simulink model "s_b16a4x512f"  (R2016b)
settings: Solver=VariableStepDiscrete  StartTime=0.0  StopTime=1  RelTol=1e-3
undefined symbols (not defined in the file): fft_stages, n_bits_ants, n_bits_xengs
libraries: xbsIndex_r4 x23057, casper_library_misc x150, xbsReplacements_r4 x9, casper_library_delays x8, xps_library x3
(part 80 of 210)

== system s_b16a4x512f/sys0/xeng/xeng_descramble/read_ctrl ==
  start : Inport
  Constant1 : xbsIndex_r4/Constant  const=ship_el_cnt  gui_display_data_type=Fixed-point  arith_type=Unsigned  n_bits=ceil(log2(ship_el_cnt+1))  bin_pt=0  preci_type=Single  exp_width=8  frac_width=24  explicit_period=on  period=1  equ=P=C  opselect=C  inp2=PCIN>>17  opr=+  inp1=P  carry=CIN  dbl_ovrd=off  block_type=constant
      settings: block_version=9.2.01
  Constant2 : xbsIndex_r4/Constant  const=ship_el_del  gui_display_data_type=Fixed-point  arith_type=Unsigned  n_bits=ship_el_del_bits  bin_pt=0  preci_type=Single  exp_width=8  frac_width=24  explicit_period=on  period=1  equ=P=C  opselect=C  inp2=PCIN>>17  opr=+  inp1=P  carry=CIN  dbl_ovrd=off  block_type=constant
      settings: block_version=9.2.01
  Gateway Out{1..2,4..8} (7 alike) : xbsIndex_r4/Gateway Out  inherit_from_input=off  hdl_port=off  rows=1  columns=1  UseAsDAC=off  DACChannel='1'  interface=None  automatic_assignment=on  address_offset=hex2dec('00')  intf_name=''  intf_description=''  timing_constraint=None  locs_specified=off  LOCs={}  io_standard={}  block_type=gatewayout
      settings: infoedit="Gateway out block.  Converts Xilinx fixed point inputs into ouputs of type Simulink integer, double, or fixed point.<P><P>Hardware notes:  In hardware these blocks become top level output ports or are discarded, depending on how they are configured."  xl_area=[0, 0, 0, 0, 0, 0, 0]  block_version=10.1.3
  Inverter3 : xbsIndex_r4/Inverter  en=off  latency=0  dbl_ovrd=off  block_type=inv
      settings: xl_area=[0, 0, 0, 0, 0, 0, 0]  block_version=9.2.01
  Logical1 : xbsIndex_r4/Logical  logical_function=AND  inputs=2  en=off  latency=0  precision=Full  arith_type=Unsigned  n_bits=8  bin_pt=2  align_bp=on  dbl_ovrd=off  block_type=logical
      settings: xl_area=[0, 0, 0, 0, 0, 0, 0]  block_version=9.2.01
  Logical7 : xbsIndex_r4/Logical  logical_function=OR  inputs=2  en=off  latency=0  precision=Full  arith_type=Unsigned  n_bits=8  bin_pt=2  align_bp=on  dbl_ovrd=off  block_type=logical
      settings: xl_area=[0, 0, 0, 0, 0, 0, 0]  block_version=9.2.01
  Register : xbsIndex_r4/Register  init=0  rst=on  en=on  dbl_ovrd=off  block_type=register
  Relational1 : xbsIndex_r4/Relational  mode=a<=b  op_type=Bool  en=off  latency=0  dbl_ovrd=off  block_type=relational
      settings: xl_area=[0, 0, 0, 0, 0, 0, 0]  block_version=9.2.01
  Relational3 : xbsIndex_r4/Relational  mode=a<=b  op_type=Bool  en=off  latency=0  dbl_ovrd=off  block_type=relational
      settings: xl_area=[0, 0, 0, 0, 0, 0, 0]  block_version=9.2.01
  Scope1 : Scope  NumInputPorts=7
  element : xbsIndex_r4/Counter  cnt_type=Free Running  cnt_to=demux_factor*num_elements+1  operation=Up  start_count=0  cnt_by_val=1  arith_type=Unsigned  n_bits=ceil(log2(ship_el_cnt+1))  bin_pt=0  load_pin=off  rst=on  en=on  explicit_period=off  period=1  use_behavioral_HDL=off  implementation=Fabric  use_rpm=on  dbl_ovrd=off  block_type=counter
      settings: xl_area=[0, 0, 0, 0, 0, 0, 0]  block_version=9.2.01
  ship_element_delay : xbsIndex_r4/Counter  cnt_type=Free Running  cnt_to=1  operation=Up  start_count=0  cnt_by_val=1  arith_type=Unsigned  n_bits=ship_el_del_bits  bin_pt=0  load_pin=off  rst=on  en=off  explicit_period=off  period=1  use_behavioral_HDL=off  implementation=Fabric  use_rpm=on  dbl_ovrd=off  block_type=counter
      settings: xl_area=[0, 0, 0, 0, 0, 0, 0]  block_version=9.2.01
  read_addr : Outport
  enable : Outport  Port=2
  wires:
  Relational3/1 -> Register/3, Register/1
  Inverter3/1 -> Logical1/2
  Register/1 -> Inverter3/1
  Logical1/1 -> element/2, Gateway Out1/1, enable/1, Gateway Out4/1
  Gateway Out2/1 -> Scope1/7
  Gateway Out1/1 -> Scope1/6
  Gateway Out8/1 -> Scope1/3
  Gateway Out6/1 -> Scope1/2
  Gateway Out5/1 -> Scope1/1
  Gateway Out4/1 -> Scope1/4
  Gateway Out7/1 -> Scope1/5
  Relational1/1 -> Logical1/1, Logical7/2, Gateway Out8/1
  Logical7/1 -> ship_element_delay/1
  ship_element_delay/1 -> Gateway Out6/1, Relational1/2
  Constant2/1 -> Relational1/1
  Constant1/1 -> Relational3/1
  element/1 -> Gateway Out2/1, read_addr/1, Relational3/2, Gateway Out7/1
  start/1 -> Register/2, element/1, Gateway Out5/1, Logical7/1

== system s_b16a4x512f/sys0/xeng/xeng_descramble/write_ctrl ==
  note: Lock onto start of new
      | valid window if previous
      | window was invalid
  note: negedge delay to
      | accomodate
      | a valid window followed
      | by an invalid window
  note: Flip this ordering to correct for
      | AxBx,AyBy,AyBx,AxBy ->AxBx,AyBy,AxBy,AyBx
  sync : Inport
  data_in : Inport  Port=2
  xeng_valid : Inport  Port=3
  window_valid : Inport  Port=4
  AddSub : xbsIndex_r4/AddSub  mode=Subtraction  use_carryin=off  use_carryout=off  en=off  latency=0  precision=Full  arith_type=Unsigned  n_bits=8  bin_pt=2  quantization=Truncate  overflow=Wrap  use_behavioral_HDL=on  hw_selection=Fabric  pipelined=off  use_rpm=on  dbl_ovrd=off  block_type=addsub
      settings: xl_area=[0, 0, 0, 0, 0, 0, 0]  block_version=9.2.01
  Constant : xbsIndex_r4/Constant  const=num_taps-1  gui_display_data_type=Fixed-point  arith_type=Unsigned  n_bits=taps_bits  bin_pt=0  preci_type=Single  exp_width=8  frac_width=24  explicit_period=on  period=1  equ=P=C  opselect=C  inp2=PCIN>>17  opr=+  inp1=P  carry=CIN  dbl_ovrd=off  block_type=constant
      settings: block_version=9.2.01
  Constant3 : xbsIndex_r4/Constant  const=ceil(num_validins*3/4)  gui_display_data_type=Fixed-point  arith_type=Unsigned  n_bits=validin_bits  bin_pt=0  preci_type=Single  exp_width=8  frac_width=24  explicit_period=on  period=1  equ=P=C  opselect=C  inp2=PCIN>>17  opr=+  inp1=P  carry=CIN  dbl_ovrd=off  block_type=constant
      settings: block_version=9.2.01
  Constant5 : xbsIndex_r4/Constant  const=0  gui_display_data_type=Fixed-point  arith_type=Unsigned  n_bits=taps_bits  bin_pt=0  preci_type=Single  exp_width=8  frac_width=24  explicit_period=on  period=1  equ=P=C  opselect=C  inp2=PCIN>>17  opr=+  inp1=P  carry=CIN  dbl_ovrd=off  block_type=constant
      settings: block_version=9.2.01
  Constant7 : xbsIndex_r4/Constant  const=num_taps-1  gui_display_data_type=Fixed-point  arith_type=Unsigned  n_bits=taps_bits  bin_pt=0  preci_type=Single  exp_width=8  frac_width=24  explicit_period=on  period=1  equ=P=C  opselect=C  inp2=PCIN>>17  opr=+  inp1=P  carry=CIN  dbl_ovrd=off  block_type=constant
      settings: block_version=9.2.01
  Convert : xbsIndex_r4/Convert  gui_display_data_type=Fixed-point  arith_type=Unsigned  n_bits=taps_bits+1  bin_pt=0  float_type=Single  exp_bits=8  fraction_bits=24  quantization=Truncate  overflow=Wrap  en=off  latency=0  pipeline=off  dbl_ovrd=off  block_type=convert
      settings: xl_area=[0, 0, 0, 0, 0, 0, 0]  block_version=9.2.01
  Counter2 : xbsIndex_r4/Counter  cnt_type=Count Limited  cnt_to=num_elements-1  operation=Up  start_count=pivot_pnt  cnt_by_val=1  arith_type=Unsigned  n_bits=ceil(log2(num_elements))  bin_pt=0  load_pin=off  rst=on  en=on  explicit_period=off  period=1  use_behavioral_HDL=off  implementation=Fabric  use_rpm=on  dbl_ovrd=off  block_type=counter
      settings: xl_area=[0, 0, 0, 0, 0, 0, 0]  block_version=9.2.01
  Counter3 : xbsIndex_r4/Counter  cnt_type=Count Limited  cnt_to=pivot_pnt-1  operation=Up  start_count=0  cnt_by_val=1  arith_type=Unsigned  n_bits=ceil(log2(num_elements))  bin_pt=0  load_pin=off  rst=on  en=on  explicit_period=off  period=1  use_behavioral_HDL=off  implementation=Fabric  use_rpm=on  dbl_ovrd=off  block_type=counter
      settings: xl_area=[0, 0, 0, 0, 0, 0, 0]  block_version=9.2.01
  Delay{,1..6} (7 alike) : xbsIndex_r4/Delay  rst=off  infoeditControl=Selection of Reset will increase slice count due to use of real FFs and instead of SRLs  en=off  latency=1  reg_retiming=on  dbl_ovrd=off  block_type=delay
  Gateway Out{1..8} (8 alike) : xbsIndex_r4/Gateway Out  inherit_from_input=off  hdl_port=off  rows=1  columns=1  UseAsDAC=off  DACChannel='1'  interface=None  automatic_assignment=on  address_offset=hex2dec('00')  intf_name=''  intf_description=''  timing_constraint=None  locs_specified=off  LOCs={}  io_standard={}  block_type=gatewayout
      settings: infoedit="Gateway out block.  Converts Xilinx fixed point inputs into ouputs of type Simulink integer, double, or fixed point.<P><P>Hardware notes:  In hardware these blocks become top level output ports or are discarded, depending on how they are configured."  xl_area=[0, 0, 0, 0, 0, 0, 0]  block_version=10.1.3
  Inverter{,1..3} (4 alike) : xbsIndex_r4/Inverter  en=off  latency=0  dbl_ovrd=off  block_type=inv
      settings: xl_area=[0, 0, 0, 0, 0, 0, 0]  block_version=9.2.01
  Logical{,2..3,5,7} (5 alike) : xbsIndex_r4/Logical  logical_function=AND  inputs=2  en=off  latency=0  precision=Full  arith_type=Unsigned  n_bits=8  bin_pt=2  align_bp=on  dbl_ovrd=off  block_type=logical
      settings: xl_area=[0, 0, 0, 0, 0, 0, 0]  block_version=9.2.01
  Logical1 : xbsIndex_r4/Logical  logical_function=OR  inputs=2  en=off  latency=0  precision=Full  arith_type=Unsigned  n_bits=8  bin_pt=2  align_bp=on  dbl_ovrd=off  block_type=logical
      settings: xl_area=[0, 0, 0, 0, 0, 0, 0]  block_version=9.2.01
  Logical4 : xbsIndex_r4/Logical  logical_function=AND  inputs=3  en=off  latency=0  precision=Full  arith_type=Unsigned  n_bits=8  bin_pt=2  align_bp=on  dbl_ovrd=off  block_type=logical
      settings: xl_area=[0, 0, 0, 0, 0, 0, 0]  block_version=9.2.01
  Logical6 : xbsIndex_r4/Logical  logical_function=OR  inputs=2  en=off  latency=0  precision=Full  arith_type=Unsigned  n_bits=8  bin_pt=2  align_bp=on  dbl_ovrd=off  block_type=logical
      settings: xl_area=[0, 0, 0, 0, 0, 0, 0]  block_version=9.2.01
  Mux : xbsIndex_r4/Mux  inputs=2  en=off  latency=0  precision=Full  arith_type="Signed  (2's comp)"  n_bits=8  bin_pt=2  quantization=Truncate  overflow=Wrap  dbl_ovrd=off  block_type=mux
      settings: xl_area=[0, 0, 0, 0, 0, 0, 0]  block_version=9.2.01
  Relational : xbsIndex_r4/Relational  mode=a=b  op_type=Bool  en=off  latency=0  dbl_ovrd=off  block_type=relational
      settings: xl_area=[0, 0, 0, 0, 0, 0, 0]  block_version=9.2.01
  Relational1 : xbsIndex_r4/Relational  mode=a>=b  op_type=Bool  en=off  latency=1  dbl_ovrd=off  block_type=relational
      settings: xl_area=[0, 0, 0, 0, 0, 0, 0]  block_version=9.2.01
  Relational3 : xbsIndex_r4/Relational  mode=a=b  op_type=Bool  en=off  latency=1  dbl_ovrd=off  block_type=relational
      settings: xl_area=[0, 0, 0, 0, 0, 0, 0]  block_version=9.2.01
  Relational4 : xbsIndex_r4/Relational  mode=a=b  op_type=Bool  en=off  latency=1  dbl_ovrd=off  block_type=relational
      settings: xl_area=[0, 0, 0, 0, 0, 0, 0]  block_version=9.2.01
  element_number : xbsIndex_r4/Counter  cnt_type=Count Limited  cnt_to=num_validins-1  operation=Up  start_count=0  cnt_by_val=1  arith_type=Unsigned  n_bits=validin_bits  bin_pt=0  load_pin=off  rst=on  en=on  explicit_period=off  period=1  use_behavioral_HDL=off  implementation=Fabric  use_rpm=on  dbl_ovrd=off  block_type=counter
      settings: xl_area=[0, 0, 0, 0, 0, 0, 0]  block_version=9.2.01
  line_number : xbsIndex_r4/Counter  cnt_type=Count Limited  cnt_to=num_ants-1  operation=Up  start_count=0  cnt_by_val=1  arith_type=Unsigned  n_bits=ant_bits  bin_pt=0  load_pin=off  rst=on  en=on  explicit_period=off  period=1  use_behavioral_HDL=off  implementation=Fabric  use_rpm=on  dbl_ovrd=off  block_type=counter
      settings: xl_area=[0, 0, 0, 0, 0, 0, 0]  block_version=9.2.01
  negate{1..4} (4 alike) : xbsIndex_r4/Negate  precision=User Defined  arith_type="Signed  (2's comp)"  n_bits=n_bits_xeng_out  bin_pt=0  quantization=Truncate  overflow=Wrap  en=off  latency=0  dbl_ovrd=off  block_type=negate
      negate1 settings: block_version=11.4
      negate2 settings: AttributesFormatString=num_ants=8  block_version=11.4
      negate3 settings: block_version=11.4
      negate4 settings: block_version=11.4
  negedge_delay : casper_library_misc/negedge_delay  pulse_len=ceil(num_ants/2)*acc_len
  posedge : casper_library_misc/edge_detect  edge=Rising  polarity=Active High  x_in=[0 0.08 0.08 0.16 0.16 0.24 0.24 0.32 0.32 0.4]  y_in="[-1 -1  1  1  1  1  1  1  1  1]"  x_out=[0.6 0.68 0.68 0.76 0.76 0.84 0.84 0.92 0.92 1]  y_out="[-1 -1  1  1 -1 -1 -1 -1 -1 -1]"
  posedge1 : casper_library_misc/edge_detect  edge=Rising  polarity=Active High  x_in=[0 0.08 0.08 0.16 0.16 0.24 0.24 0.32 0.32 0.4]  y_in="[-1 -1  1  1  1  1  1  1  1  1]"  x_out=[0.6 0.68 0.68 0.76 0.76 0.84 0.84 0.92 0.92 1]  y_out="[-1 -1  1  1 -1 -1 -1 -1 -1 -1]"
  remux : xbsIndex_r4/Concat  num_inputs=4  dbl_ovrd=off  block_type=concat
  repack{1..4} (4 alike) : casper_library_misc/ri_to_c
  sel_conj : xbsIndex_r4/Mux  inputs=2  en=off  latency=0  precision=Full  arith_type=Unsigned  n_bits=16  bin_pt=14  quantization=Truncate  overflow=Wrap  dbl_ovrd=off  block_type=mux
  slice1 : xbsIndex_r4/Slice  nbits=2*n_bits_xeng_out  boolean_output=off  mode=Lower Bit Location + Width  bit1=0  base1=MSB of Input  bit0=2*n_bits_xeng_out*3  base0=LSB of Input  dbl_ovrd=off  block_type=slice
  slice2 : xbsIndex_r4/Slice  nbits=2*n_bits_xeng_out  boolean_output=off  mode=Lower Bit Location + Width  bit1=0  base1=MSB of Input  bit0=4*n_bits_xeng_out  base0=LSB of Input  dbl_ovrd=off  block_type=slice
  slice3 : xbsIndex_r4/Slice  nbits=2*n_bits_xeng_out  boolean_output=off  mode=Lower Bit Location + Width  bit1=0  base1=MSB of Input  bit0=2*n_bits_xeng_out  base0=LSB of Input  dbl_ovrd=off  block_type=slice
  slice4 : xbsIndex_r4/Slice  nbits=2*n_bits_xeng_out  boolean_output=off  mode=Lower Bit Location + Width  bit1=0  base1=MSB of Input  bit0=0  base0=LSB of Input  dbl_ovrd=off  block_type=slice
  tap_number : xbsIndex_r4/Counter  cnt_type=Count Limited  cnt_to=num_taps-1  operation=Up  start_count=0  cnt_by_val=1  arith_type=Unsigned  n_bits=taps_bits  bin_pt=0  load_pin=off  rst=on  en=on  explicit_period=off  period=1  use_behavioral_HDL=off  implementation=Fabric  use_rpm=on  dbl_ovrd=off  block_type=counter
      settings: xl_area=[0, 0, 0, 0, 0, 0, 0]  block_version=9.2.01
  unpack{1..4} (4 alike) : casper_library_misc/c_to_ri  n_bits=n_bits_xeng_out  bin_pt=0
      settings: AttributesFormatString=25_0 r/i
  wr_ctl_debug : Scope  NumInputPorts=8
  start_readout : Outport
  write_addr : Outport  Port=2
  data_out : Outport  Port=3
  enable : Outport  Port=4
  wires:
  Delay3/1 -> [data_in]
  data_in/1 -> Delay3/1
  Delay1/1 -> [valid_in]
  sync/1 -> Delay/1
  Logical1/1 -> [rst_in]
  xeng_valid/1 -> Logical2/2
  posedge/1 -> Logical1/2
  Delay/1 -> Logical1/1
  window_valid/1 -> negedge_delay/1, posedge/1
  Logical2/1 -> Delay1/1
  negedge_delay/1 -> Logical2/1
  [data_in] -> Delay6/1
  [last_triangle] -> sel_conj/1
  repack4/1 -> remux/3
  repack3/1 -> remux/4
  Delay6/1 -> sel_conj/2, slice1/1, slice2/1, slice3/1, slice4/1
  sel_conj/1 -> data_out/1
  remux/1 -> sel_conj/3
  slice1/1 -> unpack1/1
  unpack1/1 -> repack1/1
  unpack1/2 -> negate1/1
  negate1/1 -> repack1/2
  repack1/1 -> remux/1
  slice2/1 -> unpack2/1
  unpack2/1 -> repack2/1
  unpack2/2 -> negate2/1
  negate2/1 -> repack2/2
  repack2/1 -> remux/2
  slice3/1 -> unpack3/1
  unpack3/1 -> repack3/1
  unpack3/2 -> negate3/1
  negate3/1 -> repack3/2
  slice4/1 -> unpack4/1
  unpack4/1 -> repack4/1
  unpack4/2 -> negate4/1
  negate4/1 -> repack4/2
  Delay2/1 -> [pos_cnt]
  posedge1/1 -> start_readout/1
  Relational/1 -> Logical/1, Logical6/1
  [valid_in] -> Logical6/2
  [valid_in] -> Logical/2
  [valid_in] -> element_number/2
  Delay5/1 -> [rst]
  [valid_in] -> Delay4/1
  [rst_in] -> Delay5/1
  Delay4/1 -> [valid]
  Constant7/1 -> AddSub/1
  Logical6/1 -> tap_number/2
  Constant3/1 -> Relational3/2
  element_number/1 -> Delay2/1, Relational3/1
  Logical/1 -> line_number/2
  line_number/1 -> AddSub/2
  Inverter/1 -> Logical3/2, [last_triangle]
  Convert/1 -> Relational1/1
  Relational1/1 -> Inverter/1
  Constant/1 -> Relational/1
  AddSub/1 -> Relational1/2
  tap_number/1 -> Relational/2, Relational4/2, Convert/1
  Gateway Out7/1 -> wr_ctl_debug/5
  Gateway Out4/1 -> wr_ctl_debug/4
  Gateway Out5/1 -> wr_ctl_debug/1
  Gateway Out6/1 -> wr_ctl_debug/2
  Gateway Out8/1 -> wr_ctl_debug/3
  Gateway Out1/1 -> wr_ctl_debug/6
  Gateway Out2/1 -> wr_ctl_debug/7
  [rst_in] -> tap_number/1
  [rst_in] -> line_number/1
  [rst_in] -> element_number/1
  [rst] -> Gateway Out5/1
  [last_triangle] -> Gateway Out4/1
  Constant5/1 -> Relational4/1
  [pos_cnt] -> Gateway Out1/1
  Relational4/1 -> Logical3/1
  Logical3/1 -> [blank_it]
  [blank_it] -> Inverter1/1
  [last_triangle] -> Logical4/1
  Inverter1/1 -> Logical4/2
  Logical4/1 -> Counter2/2
  Counter2/1 -> Mux/3, Gateway Out7/1
  Counter3/1 -> Mux/2
  [rst] -> Counter2/1
  [last_triangle] -> Mux/1
  Mux/1 -> write_addr/1, Gateway Out2/1
  [last_triangle] -> Inverter2/1
  [rst] -> Counter3/1
  Logical5/1 -> Counter3/2
  [valid] -> Logical4/3
  [valid] -> Logical5/1
  Inverter2/1 -> Logical5/2
  [blank_it] -> Inverter3/1
  Inverter3/1 -> Logical7/1
  [valid] -> Logical7/2
  Gateway Out3/1 -> wr_ctl_debug/8
  Logical7/1 -> enable/1, Gateway Out3/1
  Relational3/1 -> posedge1/1
  [valid] -> Gateway Out8/1
  [blank_it] -> Gateway Out6/1

== system s_b16a4x512f/sys0/xeng/xeng_descramble/x_cast ==
  in : Inport
  Concat : xbsIndex_r4/Concat  num_inputs=8  dbl_ovrd=off  block_type=concat
      settings: block_version=9.2.01
  Convert{,1..7} (8 alike) : xbsIndex_r4/Convert  gui_display_data_type=Fixed-point  arith_type="Signed  (2's comp)"  n_bits=n_bits_out  bin_pt=fix_pnt_pos  float_type=Single  exp_bits=8  fraction_bits=24  quantization=Truncate  overflow=Wrap  en=off  latency=0  pipeline=off  dbl_ovrd=off  block_type=convert
      settings: block_version=10.1.3
  Slice : xbsIndex_r4/Slice  nbits=n_bits_in  boolean_output=off  mode=Lower Bit Location + Width  bit1=0  base1=MSB of Input  bit0=bit_offsets(1)*n_bits_in  base0=LSB of Input  dbl_ovrd=off  block_type=slice
      settings: infoedit="Extracts a given range of bits from each input sample and presents it at the output.  The output type is ordinarily unsigned with binary point at zero, but can be Boolean when the slice is one bit wide.<P><P>Hardware notes: In hardware this block costs nothing."  block_version=10.1.3
  Slice1 : xbsIndex_r4/Slice  nbits=n_bits_in  boolean_output=off  mode=Lower Bit Location + Width  bit1=0  base1=MSB of Input  bit0=bit_offsets(2)*n_bits_in  base0=LSB of Input  dbl_ovrd=off  block_type=slice
      settings: infoedit="Extracts a given range of bits from each input sample and presents it at the output.  The output type is ordinarily unsigned with binary point at zero, but can be Boolean when the slice is one bit wide.<P><P>Hardware notes: In hardware this block costs nothing."  block_version=10.1.3
  Slice2 : xbsIndex_r4/Slice  nbits=n_bits_in  boolean_output=off  mode=Lower Bit Location + Width  bit1=0  base1=MSB of Input  bit0=bit_offsets(3)*n_bits_in  base0=LSB of Input  dbl_ovrd=off  block_type=slice
      settings: infoedit="Extracts a given range of bits from each input sample and presents it at the output.  The output type is ordinarily unsigned with binary point at zero, but can be Boolean when the slice is one bit wide.<P><P>Hardware notes: In hardware this block costs nothing."  block_version=10.1.3
  Slice3 : xbsIndex_r4/Slice  nbits=n_bits_in  boolean_output=off  mode=Lower Bit Location + Width  bit1=0  base1=MSB of Input  bit0=bit_offsets(4)*n_bits_in  base0=LSB of Input  dbl_ovrd=off  block_type=slice
      settings: infoedit="Extracts a given range of bits from each input sample and presents it at the output.  The output type is ordinarily unsigned with binary point at zero, but can be Boolean when the slice is one bit wide.<P><P>Hardware notes: In hardware this block costs nothing."  block_version=10.1.3
  Slice4 : xbsIndex_r4/Slice  nbits=n_bits_in  boolean_output=off  mode=Lower Bit Location + Width  bit1=0  base1=MSB of Input  bit0=bit_offsets(5)*n_bits_in  base0=LSB of Input  dbl_ovrd=off  block_type=slice
      settings: infoedit="Extracts a given range of bits from each input sample and presents it at the output.  The output type is ordinarily unsigned with binary point at zero, but can be Boolean when the slice is one bit wide.<P><P>Hardware notes: In hardware this block costs nothing."  block_version=10.1.3
  Slice5 : xbsIndex_r4/Slice  nbits=n_bits_in  boolean_output=off  mode=Lower Bit Location + Width  bit1=0  base1=MSB of Input  bit0=bit_offsets(6)*n_bits_in  base0=LSB of Input  dbl_ovrd=off  block_type=slice
      settings: infoedit="Extracts a given range of bits from each input sample and presents it at the output.  The output type is ordinarily unsigned with binary point at zero, but can be Boolean when the slice is one bit wide.<P><P>Hardware notes: In hardware this block costs nothing."  block_version=10.1.3
  Slice6 : xbsIndex_r4/Slice  nbits=n_bits_in  boolean_output=off  mode=Lower Bit Location + Width  bit1=0  base1=MSB of Input  bit0=bit_offsets(7)*n_bits_in  base0=LSB of Input  dbl_ovrd=off  block_type=slice
      settings: infoedit="Extracts a given range of bits from each input sample and presents it at the output.  The output type is ordinarily unsigned with binary point at zero, but can be Boolean when the slice is one bit wide.<P><P>Hardware notes: In hardware this block costs nothing."  block_version=10.1.3
  Slice7 : xbsIndex_r4/Slice  nbits=n_bits_in  boolean_output=off  mode=Lower Bit Location + Width  bit1=0  base1=MSB of Input  bit0=bit_offsets(8)*n_bits_in  base0=LSB of Input  dbl_ovrd=off  block_type=slice
      settings: infoedit="Extracts a given range of bits from each input sample and presents it at the output.  The output type is ordinarily unsigned with binary point at zero, but can be Boolean when the slice is one bit wide.<P><P>Hardware notes: In hardware this block costs nothing."  block_version=10.1.3
  force_re{,1,4,6,8,10,12,14} (8 alike) : xbsIndex_r4/Reinterpret  force_arith_type=on  arith_type="Signed  (2's comp)"  force_bin_pt=on  bin_pt=fix_pnt_pos  block_type=reinterpret
      settings: infoedit="Changes signal type without altering the binary representation.   You can changed the signal between signed and unsigned, and relocate the binary point.<P><P>Hardware notes: In hardware this block costs nothing.<P><P>Example:  Suppose the input is 6 bits wide, signed, with 2 fractional bits, and the output is forced to unsigned with 0 fractional bits.  Then an input of -2.0 (1110.00 in binary 2's complement) becomes an output of 56 (111000 in binary)."  block_version=9.1.01
  force_re{2..3,5,7,9,11,13,15} (8 alike) : xbsIndex_r4/Reinterpret  force_arith_type=on  arith_type=Unsigned  force_bin_pt=on  bin_pt=0  block_type=reinterpret
      settings: infoedit="Changes signal type without altering the binary representation.   You can changed the signal between signed and unsigned, and relocate the binary point.<P><P>Hardware notes: In hardware this block costs nothing.<P><P>Example:  Suppose the input is 6 bits wide, signed, with 2 fractional bits, and the output is forced to unsigned with 0 fractional bits.  Then an input of -2.0 (1110.00 in binary 2's complement) becomes an output of 56 (111000 in binary)."  block_version=9.1.01
  out : Outport
  wires:
  force_re15/1 -> Concat/8
  force_re13/1 -> Concat/7
  force_re11/1 -> Concat/6
  force_re9/1 -> Concat/5
  force_re7/1 -> Concat/4
  force_re5/1 -> Concat/3
  Slice7/1 -> force_re14/1
  force_re14/1 -> Convert7/1
  Convert7/1 -> force_re15/1
  Slice6/1 -> force_re12/1
  force_re12/1 -> Convert6/1
  Convert6/1 -> force_re13/1
  Slice5/1 -> force_re10/1
  force_re10/1 -> Convert5/1
  Convert5/1 -> force_re11/1
  Slice4/1 -> force_re8/1
  force_re8/1 -> Convert4/1
  Convert4/1 -> force_re9/1
  Slice3/1 -> force_re6/1
  force_re6/1 -> Convert3/1
  Convert3/1 -> force_re7/1
  Slice2/1 -> force_re4/1
  force_re4/1 -> Convert2/1
  Convert2/1 -> force_re5/1
  force_re3/1 -> Concat/2
  Slice1/1 -> force_re1/1
  Concat/1 -> out/1
  in/1 -> Slice1/1, Slice2/1, Slice3/1, Slice4/1, Slice5/1, Slice7/1, Slice6/1, Slice/1
  Slice/1 -> force_re/1
  force_re1/1 -> Convert1/1
  force_re/1 -> Convert/1
  Convert1/1 -> force_re3/1
  Convert/1 -> force_re2/1
  force_re2/1 -> Concat/1

== system s_b16a4x512f/sys1/bf/fbf/apply_beam_weights ==
  note: The same coefficient
      | is kept for each 'stack'
      | of input values
  note: Xilinx addresses words in a compound
      | word as 0 in the LS word. We want it
      | the other way so we reorder the data
      | on the way in and then undo the
      | reordering on the way out again
  synci : Inport
  din : Inport  Port=2
  den : Inport  Port=3
  misci : Inport  Port=4
  index : Inport  Port=5
  vali : Inport  Port=6
  we : Inport  Port=7
  Concat : xbsIndex_r4/Concat  num_inputs=3  dbl_ovrd=off  block_type=concat
  Constant1 : xbsIndex_r4/Constant  const=0  gui_display_data_type=Fixed-point  arith_type=Boolean  n_bits=1  bin_pt=0  preci_type=Single  exp_width=8  frac_width=24  explicit_period=off  period=1  equ=P=C  opselect=C  inp2=PCIN>>17  opr=+  inp1=P  carry=CIN  dbl_ovrd=off  block_type=constant
      settings: block_version=11.4
  Slice : xbsIndex_r4/Slice  nbits=1  boolean_output=on  mode=Upper Bit Location + Width  bit1=-1  base1=MSB of Input  bit0=0  base0=LSB of Input  dbl_ovrd=off  block_type=slice
  Slice1 : xbsIndex_r4/Slice  nbits=1  boolean_output=off  mode=Two Bit Locations  bit1=-2  base1=MSB of Input  bit0=0  base0=LSB of Input  dbl_ovrd=off  block_type=slice
  Slice2 : xbsIndex_r4/Slice  nbits=1  boolean_output=on  mode=Upper Bit Location + Width  bit1=0  base1=MSB of Input  bit0=0  base0=LSB of Input  dbl_ovrd=off  block_type=slice
  add_gen : xbsIndex_r4/Counter  cnt_type=Free Running  cnt_to=Inf  operation=Up  start_count=0  cnt_by_val=1  arith_type=Unsigned  n_bits=vec_bits+stack_bits  bin_pt=0  load_pin=off  rst=on  en=on  explicit_period=on  period=1  use_behavioral_HDL=off  implementation=Fabric  dbl_ovrd=off  block_type=counter
      settings: block_version=11.4
  bus_convert : Subsystem  AncestorBlock=casper_library_bus/bus_convert  mask(bus_convert){n_bits_in=repmat(n_bits_coeff+n_bits_in+1, 1, 2^stream_bits), bin_pt_in=bin_pt_coeff+bin_pt_in, cmplx=on, n_bits_out=n_bits_out, bin_pt_out=bin_pt_out, quantization=quantization, overflow=overflow, latency=conv_latency, of=off, misc=on}
      mask prompts: n_bits_in "input bit widths"; bin_pt_in "input binary points"; cmplx "input complex"; n_bits_out "output bit widths"; bin_pt_out "output binary points"; quantization "quantization strategy (Truncate=0, Round  (unbiased: +/- Inf)=1, Round (unbiased: Even Values)=2)"; overflow "overflow strategy (Wrap=0, Saturate=1, Flag as error=2)"; of "overflow indication"; misc "misc support"
      mask help: Convert components of busses
      mask init: same as s_b16a4x512f/sys0/31->32
  bus_mult : Subsystem  AncestorBlock=casper_library_bus/bus_mult  mask(bus_mult){n_bits_a=repmat(n_bits_in, 1, 2^stream_bits), bin_pt_a=bin_pt_in, type_a=type_in, cmplx_a=on, n_bits_b=repmat(n_bits_coeff, 1, 2^stream_bits), bin_pt_b=bin_pt_coeff, type_b=type_coeff, cmplx_b=off, n_bits_out=n_bits_coeff+n_bits_in+1, bin_pt_out=bin_pt_coeff+bin_pt_in, type_out=type_out, quantization=0, overflow=0, mult_latency=mult_latency, add_latency=2, conv_latency=0, max_fanout=2, fan_latency=1, multiplier_implementation=embedded multiplier core, misc=on}
      mask prompts: n_bits_a "a input bit widths"; bin_pt_a "a input binary points"; type_a "a input type (Unsigned=0, Signed=1)"; cmplx_a "a input complex"; n_bits_b "b input bit widths"; bin_pt_b "b input binary points"; type_b "b input type (Unsigned=0, Signed=1)"; cmplx_b "b input complex"; n_bits_out "output bit widths"; bin_pt_out "output binary points"; type_out "output type (Unsigned=0, Signed=1)"; quantization "quantization strategy (Truncate=0, Round  (unbiased: +/- Inf)=1)"; overflow "overflow strategy (Wrap=0, Saturate=1, Flag as error=2)"; mult_latency "multiplier latency"; add_latency "adder latency"; conv_latency "convert latency"; max_fanout "limit fanout to ?"; fan_latency "fanout register latency"; multiplier_implementation "multiplier implementation"; misc "misc support"
      mask help: Multiply components of two busses
      mask init: same as s_b16a4x512f/sys0/bf/fbf/apply_beam_weights/bus_mult
      mask TypeOptions multiplier_implementation: behavioral HDL | standard core | embedded multiplier core
  coeffs : xbsIndex_r4/Dual Port RAM  depth=2^(vec_bits+stream_bits)  initVector=repmat(real(init_val)*2^(bin_pt_coeff),1,2^(vec_bits+stream_bits))  distributed_mem=Block RAM  init_a=0  init_b=0  rst_a=off  rst_b=off  en_a=off  en_b=off  latency=bram_latency  write_mode_A=Read After Write  write_mode_B=Read After Write  optimize=Area  dbl_ovrd=off  block_type=dpram
      settings: block_version=11.4
  ddin : xbsIndex_r4/Delay  rst=off  infoeditControl=Selection of Reset will increase slice count due to use of real FFs and instead of SRLs  en=off  latency=bram_latency  reg_retiming=off  dbl_ovrd=off  block_type=delay
      settings: block_version=11.4
  ddin1 : xbsIndex_r4/Delay  rst=off  infoeditControl=Selection of Reset will increase slice count due to use of real FFs and instead of SRLs  en=off  latency=bram_latency  reg_retiming=off  dbl_ovrd=off  block_type=delay
      settings: block_version=11.4
  dinb : xbsIndex_r4/Constant  const=0  gui_display_data_type=Fixed-point  arith_type=Unsigned  n_bits=n_bits_coeff*2^stream_bits  bin_pt=0  preci_type=Single  exp_width=8  frac_width=24  explicit_period=off  period=1  equ=P=C  opselect=C  inp2=PCIN>>17  opr=+  inp1=P  carry=CIN  dbl_ovrd=off  block_type=constant
      settings: block_version=11.4
  munge_in : Subsystem  AncestorBlock=casper_library_flow_control/munge  mask(munge){divisions=2^stream_bits, div_size=repmat(n_bits_in*2, 1, 2^stream_bits), order=max(0,2^stream_bits-1):-1:0, arith_type_out=Unsigned, bin_pt_out=0}
      mask prompts: divisions "Number of divisions"; div_size "Division size (bits)"; order "Division packing order"; arith_type_out "Output arithmetic type"; bin_pt_out "Output binary point"
      mask help: Splits an input bus into the specified number of divisions and then recombines them in the order specified (most significant division = 0,least = number divisions-1)
      mask init:
      | munge_init(gcb, ...
      |     'divisions', divisions, ...
      |     'div_size', div_size, ...
      |     'order', order, ...
      |     'arith_type_out', arith_type_out, ...
      |     'bin_pt_out', bin_pt_out);
      settings: AttributesFormatString=|
      | split:[16 16]
      | join:[1 0]
      | Unsigned [32,0]
      mask TypeOptions arith_type_out: Unsigned | Signed  (2's comp) | Floating-point
  munge_out : Subsystem  AncestorBlock=casper_library_flow_control/munge  mask(munge){divisions=2^stream_bits, div_size=repmat(n_bits_out*2, 1, 2^stream_bits), order=max(0,2^stream_bits-1):-1:0, arith_type_out=Unsigned, bin_pt_out=0}
      mask prompts: divisions "Number of divisions"; div_size "Division size (bits)"; order "Division packing order"; arith_type_out "Output arithmetic type"; bin_pt_out "Output binary point"
      mask help: Splits an input bus into the specified number of divisions and then recombines them in the order specified (most significant division = 0,least = number divisions-1)
      mask init:
      | munge_init(gcb, ...
      |     'divisions', divisions, ...
      |     'div_size', div_size, ...
      |     'order', order, ...
      |     'arith_type_out', arith_type_out, ...
      |     'bin_pt_out', bin_pt_out);
      settings: AttributesFormatString=|
      | split:[50 50]
      | join:[1 0]
      | Unsigned [100,0]
      mask TypeOptions arith_type_out: Unsigned | Signed  (2's comp) | Floating-point
  vector : xbsIndex_r4/Slice  nbits=vec_bits  boolean_output=off  mode=Lower Bit Location + Width  bit1=0  base1=MSB of Input  bit0=stack_bits  base0=LSB of Input  dbl_ovrd=off  block_type=slice
  we_slice : xbsIndex_r4/Slice  nbits=1  boolean_output=on  mode=Lower Bit Location + Width  bit1=0  base1=MSB of Input  bit0=0  base0=LSB of Input  dbl_ovrd=off  block_type=slice
  synco : Outport
  dout : Outport  Port=2
  eno : Outport  Port=3
  misco : Outport  Port=4
  valo : Outport  Port=5
  wires:
  add_gen/1 -> vector/1
  vector/1 -> coeffs/4
  dinb/1 -> coeffs/5
  we_slice/1 -> coeffs/3
  Constant1/1 -> coeffs/6
  coeffs/1 -> valo/1
  index/1 -> coeffs/1
  den/1 -> add_gen/2, Concat/2
  din/1 -> ddin/1
  we/1 -> we_slice/1
  synci/1 -> Concat/1, add_gen/1
  ddin/1 -> munge_in/1(din)
  coeffs/2 -> bus_mult/2(b)
  Concat/1 -> ddin1/1
  ddin1/1 -> bus_mult/3(misci)
  Slice/1 -> eno/1
  Slice1/1 -> misco/1
  bus_mult/1(a*b) -> bus_convert/1(din)
  bus_mult/2(misco) -> bus_convert/2(misci)
  bus_convert/1(dout) -> munge_out/1(din)
  bus_convert/2(misco) -> Slice1/1, Slice2/1, Slice/1
  misci/1 -> Concat/3
  Slice2/1 -> synco/1
  vali/1 -> coeffs/2
  munge_in/1(dout) -> bus_mult/1(a)
  munge_out/1(dout) -> dout/1

== system s_b16a4x512f/sys1/bf/fbf/bus_expand ==
  bus_in : Inport
  reinterpret{1..4} (4 alike) : xbsIndex_r4/Reinterpret  force_arith_type=on  arith_type="Signed  (2's comp)"  force_bin_pt=on  bin_pt=7  block_type=reinterpret
      settings: infoedit="Changes signal type without altering the binary representation.   You can changed the signal between signed and unsigned, and relocate the binary point.<br><br>Hardware notes: In hardware this block costs nothing.<br><br>Example:  Suppose the input is 6 bits wide, signed, with 2 fractional bits, and the output is forced to unsigned with 0 fractional bits.  Then an input of -2.0 (1110.00 in binary 2's complement) becomes an output of 56 (111000 in binary)."
  slice1 : xbsIndex_r4/Slice  nbits=8  boolean_output=off  mode=Upper Bit Location + Width  bit1=-24  base1=MSB of Input  bit0=0  base0=LSB of Input  dbl_ovrd=off  block_type=slice
  slice2 : xbsIndex_r4/Slice  nbits=8  boolean_output=off  mode=Upper Bit Location + Width  bit1=-16  base1=MSB of Input  bit0=0  base0=LSB of Input  dbl_ovrd=off  block_type=slice
  slice3 : xbsIndex_r4/Slice  nbits=8  boolean_output=off  mode=Upper Bit Location + Width  bit1=-8  base1=MSB of Input  bit0=0  base0=LSB of Input  dbl_ovrd=off  block_type=slice
  slice4 : xbsIndex_r4/Slice  nbits=8  boolean_output=off  mode=Upper Bit Location + Width  bit1=0  base1=MSB of Input  bit0=0  base0=LSB of Input  dbl_ovrd=off  block_type=slice
  msb_out4 : Outport
  out3 : Outport  Port=2
  out2 : Outport  Port=3
  lsb_out1 : Outport  Port=4
  wires:
  bus_in/1 -> slice4/1, slice3/1, slice2/1, slice1/1
  slice4/1 -> reinterpret4/1
  reinterpret4/1 -> msb_out4/1
  slice3/1 -> reinterpret3/1
  reinterpret3/1 -> out3/1
  slice2/1 -> reinterpret2/1
  reinterpret2/1 -> out2/1
  slice1/1 -> reinterpret1/1
  reinterpret1/1 -> lsb_out1/1

== system s_b16a4x512f/sys1/bf/fbf/bus_expand1 ==
  bus_in : Inport
  reinterpret{1..4} (4 alike) : xbsIndex_r4/Reinterpret  force_arith_type=on  arith_type="Signed  (2's comp)"  force_bin_pt=on  bin_pt=16  block_type=reinterpret
      settings: infoedit="Changes signal type without altering the binary representation.   You can changed the signal between signed and unsigned, and relocate the binary point.<br><br>Hardware notes: In hardware this block costs nothing.<br><br>Example:  Suppose the input is 6 bits wide, signed, with 2 fractional bits, and the output is forced to unsigned with 0 fractional bits.  Then an input of -2.0 (1110.00 in binary 2's complement) becomes an output of 56 (111000 in binary)."
  slice1 : xbsIndex_r4/Slice  nbits=25  boolean_output=off  mode=Upper Bit Location + Width  bit1=-75  base1=MSB of Input  bit0=0  base0=LSB of Input  dbl_ovrd=off  block_type=slice
  slice2 : xbsIndex_r4/Slice  nbits=25  boolean_output=off  mode=Upper Bit Location + Width  bit1=-50  base1=MSB of Input  bit0=0  base0=LSB of Input  dbl_ovrd=off  block_type=slice
  slice3 : xbsIndex_r4/Slice  nbits=25  boolean_output=off  mode=Upper Bit Location + Width  bit1=-25  base1=MSB of Input  bit0=0  base0=LSB of Input  dbl_ovrd=off  block_type=slice
  slice4 : xbsIndex_r4/Slice  nbits=25  boolean_output=off  mode=Upper Bit Location + Width  bit1=0  base1=MSB of Input  bit0=0  base0=LSB of Input  dbl_ovrd=off  block_type=slice
  msb_out4 : Outport
  out3 : Outport  Port=2
  out2 : Outport  Port=3
  lsb_out1 : Outport  Port=4
  wires:
  bus_in/1 -> slice4/1, slice3/1, slice2/1, slice1/1
  slice4/1 -> reinterpret4/1
  reinterpret4/1 -> msb_out4/1
  slice3/1 -> reinterpret3/1
  reinterpret3/1 -> out3/1
  slice2/1 -> reinterpret2/1
  reinterpret2/1 -> out2/1
  slice1/1 -> reinterpret1/1
  reinterpret1/1 -> lsb_out1/1

== system s_b16a4x512f/sys1/bf/fbf/combine ==
  note: *  accumulator that takes values for all
      | beams for bunch of time for associated antenna
      | * outputs values when all antennae
      | accounted for
      | * excludes if bad bit high
  synci : Inport
  data : Inport  Port=2
  den : Inport  Port=3
  bad : Inport  Port=4
  timei : Inport  Port=5
  misci : Inport  Port=6
  Concat : xbsIndex_r4/Concat  num_inputs=2  dbl_ovrd=off  block_type=concat
  acc : Subsystem  mask{stream_bits=stream_bits, stack_bits=stack_bits, n_bits_in=n_bits_in, bin_pt_in=bin_pt_in, n_bits_accum=n_bits_accum, bram_latency=bram_latency, add_latency=add_latency}
      mask prompts: stream_bits "input streams (2^?)"; stack_bits "stacking factor (2^?)"; n_bits_in "data bits in"; bin_pt_in "binary point in"; n_bits_accum "accumulator bits"; bram_latency "bram latency"; add_latency "add latency"
      mask init: same as s_b16a4x512f/sys0/bf/fbf/combine/acc
  acc_ctrl : Subsystem  mask{ant_bits=ant_bits, stream_bits=stream_bits, freq_bits=freq_bits, stack_bits=stack_bits, bram_latency=bram_latency}
      mask prompts: ant_bits "antennas (2^?)"; stream_bits "input streams (2^?)"; freq_bits "frequencies (2^?)"; stack_bits "stacking factor (2^?)"; bram_latency "bram latency"
  misc_slc : xbsIndex_r4/Slice  nbits=0  boolean_output=off  mode=Two Bit Locations  bit1=-timestamp_bits  base1=MSB of Input  bit0=0  base0=LSB of Input  dbl_ovrd=off  block_type=slice
  time_slc : xbsIndex_r4/Slice  nbits=timestamp_bits  boolean_output=off  mode=Upper Bit Location + Width  bit1=0  base1=MSB of Input  bit0=0  base0=LSB of Input  dbl_ovrd=off  block_type=slice
  synco : Outport
  sum : Outport  Port=2
  eno : Outport  Port=3
  timeo : Outport  Port=4
  misco : Outport  Port=5
  wires:
  acc/1(synco) -> synco/1
  acc_ctrl/1(synco) -> acc/1(synci)
  misc_slc/1 -> misco/1
  time_slc/1 -> timeo/1
  acc/4(misc_o) -> misc_slc/1, time_slc/1
  Concat/1 -> acc/6(misc_in)
  acc_ctrl/7(misco) -> Concat/2
  acc_ctrl/6(timeo) -> Concat/1
  acc_ctrl/5(dump) -> acc/5(dump)
  acc_ctrl/4(dvalid) -> acc/4(dvalid)
  bad/1 -> acc_ctrl/4(badi)
  timei/1 -> acc_ctrl/5(timei)
  acc_ctrl/3(en) -> acc/3(en)
  acc_ctrl/2(dout) -> acc/2(dat)
  synci/1 -> acc_ctrl/1(synci)
  den/1 -> acc_ctrl/3(den)
  acc/2(dato) -> sum/1
  data/1 -> acc_ctrl/2(din)
  acc/3(valid) -> eno/1
  misci/1 -> acc_ctrl/6(misci)

== system s_b16a4x512f/sys1/bf/fbf/duplicate ==
  synci : Inport
  eni : Inport  Port=2
  di : Inport  Port=3
  badi : Inport  Port=4
  timei : Inport  Port=5
  misci : Inport  Port=6
  sim_ld : Inport  Port=7
  sim_type : Inport  Port=8
  Convert1 : xbsIndex_r4/Convert  gui_display_data_type=Fixed-point  arith_type=Unsigned  n_bits=n_bits_in*2  bin_pt=0  float_type=Single  exp_bits=8  fraction_bits=24  quantization=Truncate  overflow=Wrap  en=off  latency=0  pipeline=off  dbl_ovrd=off  block_type=convert
      settings: block_version=11.4
  Counter : xbsIndex_r4/Counter  cnt_type=Free Running  cnt_to=inf  operation=Up  start_count=0  cnt_by_val=1  arith_type="Signed  (2's comp)"  n_bits=stack_bits+ant_bits+freq_bits  bin_pt=0  load_pin=off  rst=on  en=on  explicit_period=on  period=1  use_behavioral_HDL=off  implementation=Fabric  dbl_ovrd=off  block_type=counter
      settings: block_version=11.4
  Delay{,1..3,5} (5 alike) : xbsIndex_r4/Delay  rst=off  infoeditControl=Selection of Reset will increase slice count due to use of real FFs and instead of SRLs  en=off  latency=1  reg_retiming=off  dbl_ovrd=off  block_type=delay
      Delay settings: infoedit=Hardware notes: A delay line is a chain, each link of which is an SRL16 or SRL32 followed by a flip-flop.  block_version=11.4
      Delay1 settings: block_version=11.4
      Delay2 settings: block_version=11.4
      Delay3 settings: block_version=11.4
      Delay5 settings: block_version=11.4
  Mux : xbsIndex_r4/Mux  inputs=2  en=off  latency=1  precision=Full  arith_type=Unsigned  n_bits=16  bin_pt=14  quantization=Truncate  overflow=Wrap  dbl_ovrd=off  block_type=mux
      settings: block_version=11.4
  Register1 : xbsIndex_r4/Register  init=0  rst=off  en=on  dbl_ovrd=off  block_type=register
      settings: block_version=11.4
  Slice : xbsIndex_r4/Slice  nbits=freq_bits  boolean_output=off  mode=Upper Bit Location + Width  bit1=0  base1=MSB of Input  bit0=0  base0=LSB of Input  dbl_ovrd=off  block_type=slice
  beam_replicate : Subsystem  AncestorBlock=casper_library_bus/bus_replicate  mask(bus_replicate){replication=2^beam_bits, latency=0, misc=off, implementation=core}
      mask prompts: replication "replication factor"; misc "misc support"; implementation "delay implementation"
      mask help: Output bus formed by replicating input bus a number of times
      mask init:
      | bus_replicate_init(gcb, ...
      |     'replication', replication, ...
      |     'latency', latency, ...
      |     'implementation', implementation, ...
      |     'misc', misc);
      mask TypeOptions implementation: core | behavioral
  pol_replicate : Subsystem  AncestorBlock=casper_library_bus/bus_replicate  mask(bus_replicate){replication=2^polarisation_bits, latency=0, misc=off, implementation=core}
      mask prompts: replication "replication factor"; misc "misc support"; implementation "delay implementation"
      mask help: Output bus formed by replicating input bus a number of times
      mask init:
      | bus_replicate_init(gcb, ...
      |     'replication', replication, ...
      |     'latency', latency, ...
      |     'implementation', implementation, ...
      |     'misc', misc);
      mask TypeOptions implementation: core | behavioral
  synco : Outport
  do : Outport  Port=2
  eno : Outport  Port=3
  bado : Outport  Port=4
  timeo : Outport  Port=5
  misco : Outport  Port=6
  wires:
  synci/1 -> Delay/1, Counter/1
  eni/1 -> Counter/2, Delay2/1
  badi/1 -> Delay3/1
  misci/1 -> Delay5/1
  timei/1 -> Delay1/1
  Delay/1 -> synco/1
  Delay3/1 -> bado/1
  Delay5/1 -> misco/1
  Delay1/1 -> timeo/1
  sim_ld/1 -> Register1/2
  sim_type/1 -> Register1/1
  beam_replicate/1(out) -> do/1
  Mux/1 -> beam_replicate/1(in)
  Register1/1 -> Mux/1
  di/1 -> Mux/2
  Counter/1 -> Slice/1
  pol_replicate/1(out) -> Mux/3
  Slice/1 -> Convert1/1
  Convert1/1 -> pol_replicate/1(in)
  Delay2/1 -> eno/1

== system s_b16a4x512f/sys1/bf/fbf/pipeline1 ==
  d : Inport
  Register0 : xbsIndex_r4/Register  init=0  rst=off  en=off  dbl_ovrd=off  block_type=register
      settings: block_version=11.4
  Register1 : xbsIndex_r4/Register  init=0  rst=off  en=off  dbl_ovrd=off  block_type=register
      settings: block_version=11.4
  q : Outport
  wires:
  Register1/1 -> q/1
  d/1 -> Register0/1
  Register0/1 -> Register1/1

== system s_b16a4x512f/sys1/bf/fbf/pipeline10 ==
  d : Inport
  Register0 : xbsIndex_r4/Register  init=0  rst=off  en=off  dbl_ovrd=off  block_type=register
      settings: block_version=11.4
  Register1 : xbsIndex_r4/Register  init=0  rst=off  en=off  dbl_ovrd=off  block_type=register
      settings: block_version=11.4
  q : Outport
  wires:
  Register0/1 -> Register1/1
  d/1 -> Register0/1
  Register1/1 -> q/1

== system s_b16a4x512f/sys1/bf/fbf/pipeline11 ==
  d : Inport
  Register0 : xbsIndex_r4/Register  init=0  rst=off  en=off  dbl_ovrd=off  block_type=register
      settings: block_version=11.4
  Register1 : xbsIndex_r4/Register  init=0  rst=off  en=off  dbl_ovrd=off  block_type=register
      settings: block_version=11.4
  q : Outport
  wires:
  Register1/1 -> q/1
  d/1 -> Register0/1
  Register0/1 -> Register1/1

== system s_b16a4x512f/sys1/bf/fbf/pipeline12 ==
  d : Inport
  Register0 : xbsIndex_r4/Register  init=0  rst=off  en=off  dbl_ovrd=off  block_type=register
      settings: block_version=11.4
  Register1 : xbsIndex_r4/Register  init=0  rst=off  en=off  dbl_ovrd=off  block_type=register
      settings: block_version=11.4
  q : Outport
  wires:
  Register0/1 -> Register1/1
  d/1 -> Register0/1
  Register1/1 -> q/1

== system s_b16a4x512f/sys1/bf/fbf/pipeline13 ==
  d : Inport
  Register0 : xbsIndex_r4/Register  init=0  rst=off  en=off  dbl_ovrd=off  block_type=register
      settings: block_version=11.4
  Register1 : xbsIndex_r4/Register  init=0  rst=off  en=off  dbl_ovrd=off  block_type=register
      settings: block_version=11.4
  q : Outport
  wires:
  Register1/1 -> q/1
  d/1 -> Register0/1
  Register0/1 -> Register1/1

== system s_b16a4x512f/sys1/bf/fbf/pipeline14 ==
  d : Inport
  Register0 : xbsIndex_r4/Register  init=0  rst=off  en=off  dbl_ovrd=off  block_type=register
      settings: block_version=11.4
  Register1 : xbsIndex_r4/Register  init=0  rst=off  en=off  dbl_ovrd=off  block_type=register
      settings: block_version=11.4
  q : Outport
  wires:
  Register0/1 -> Register1/1
  d/1 -> Register0/1
  Register1/1 -> q/1

== system s_b16a4x512f/sys1/bf/fbf/pipeline15 ==
  d : Inport
  Register0 : xbsIndex_r4/Register  init=0  rst=off  en=off  dbl_ovrd=off  block_type=register
      settings: block_version=11.4
  Register1 : xbsIndex_r4/Register  init=0  rst=off  en=off  dbl_ovrd=off  block_type=register
      settings: block_version=11.4
  q : Outport
  wires:
  Register0/1 -> Register1/1
  d/1 -> Register0/1
  Register1/1 -> q/1

== system s_b16a4x512f/sys1/bf/fbf/pipeline16 ==
  d : Inport
  Register0 : xbsIndex_r4/Register  init=0  rst=off  en=off  dbl_ovrd=off  block_type=register
      settings: block_version=11.4
  Register1 : xbsIndex_r4/Register  init=0  rst=off  en=off  dbl_ovrd=off  block_type=register
      settings: block_version=11.4
  q : Outport
  wires:
  Register1/1 -> q/1
  d/1 -> Register0/1
  Register0/1 -> Register1/1

== system s_b16a4x512f/sys1/bf/fbf/pipeline2 ==
  d : Inport
  Register0 : xbsIndex_r4/Register  init=0  rst=off  en=off  dbl_ovrd=off  block_type=register
      settings: block_version=11.4
  Register1 : xbsIndex_r4/Register  init=0  rst=off  en=off  dbl_ovrd=off  block_type=register
      settings: block_version=11.4
  q : Outport
  wires:
  Register0/1 -> Register1/1
  d/1 -> Register0/1
  Register1/1 -> q/1

== system s_b16a4x512f/sys1/bf/fbf/pipeline3 ==
  d : Inport
  Register0 : xbsIndex_r4/Register  init=0  rst=off  en=off  dbl_ovrd=off  block_type=register
      settings: block_version=11.4
  Register1 : xbsIndex_r4/Register  init=0  rst=off  en=off  dbl_ovrd=off  block_type=register
      settings: block_version=11.4
  q : Outport
  wires:
  Register1/1 -> q/1
  d/1 -> Register0/1
  Register0/1 -> Register1/1

== system s_b16a4x512f/sys1/bf/fbf/pipeline8 ==
  d : Inport
  Register0 : xbsIndex_r4/Register  init=0  rst=off  en=off  dbl_ovrd=off  block_type=register
      settings: block_version=11.4
  Register1 : xbsIndex_r4/Register  init=0  rst=off  en=off  dbl_ovrd=off  block_type=register
      settings: block_version=11.4
  q : Outport
  wires:
  Register1/1 -> q/1
  d/1 -> Register0/1
  Register0/1 -> Register1/1

== system s_b16a4x512f/sys1/bf/fbf/pipeline9 ==
  d : Inport
  Register0 : xbsIndex_r4/Register  init=0  rst=off  en=off  dbl_ovrd=off  block_type=register
      settings: block_version=11.4
  Register1 : xbsIndex_r4/Register  init=0  rst=off  en=off  dbl_ovrd=off  block_type=register
      settings: block_version=11.4
  q : Outport
  wires:
  Register0/1 -> Register1/1
  d/1 -> Register0/1
  Register1/1 -> q/1
